simulink model "Shaddad_NavFusion"  (R2026b)
undefined symbols (not defined in the file): P, Ts
libraries: simulink x18, robotcorelib x4, ros2lib x3, mspfiltlib x2
(part 2 of 2)

== matlab function Shaddad_NavFusion/NavGate ==
  settings: updateMethod=DISCRETE  sampleTime=Ts.nav  description=Innovation gating and time-varying R of the navigation EKF (subsystems/sensors/sens_nav_gate.m).
  data: xP input; en output; PP input; uP input; QP input; rst input; z1 input; z2 input; z3 input; z4 input; z5 input; avail input; accG input; s3 input; C5 input; u1 input; u2 input; u3 input; u4 input; u5 input; fix input; R1 output; R2 output; R3 output; R4 output; R5 output; nis output; rej output; prm parameter
function [en, R1, R2, R3, R4, R5, nis, rej] = fcn(xP, PP, uP, QP, rst, z1, z2, z3, z4, z5, avail, accG, s3, C5, u1, u2, u3, u4, u5, fix, prm)
[en, R1, R2, R3, R4, R5, nis, rej] = sens_nav_gate(xP, PP, uP, QP, rst, z1, z2, z3, z4, z5, avail, accG, s3, C5, u1, u2, u3, u4, u5, fix, prm);
